simulink model "tg9"  (R2022a)
settings: Solver=ode15s  StartTime=0.0  StopTime=10  MaxStep=0.01  RelTol=1e-3
InitFcn:
  | mecha_param2
  | control_param0
values from neighbouring files (symbols this model uses):
  b0 = 0    [sim_IMMC.m]
  b1 = 1    [sim_IMMC.m]
  back0 = 0    [sim_IMMC.m]
  back1 = 0    [sim_IMMC.m]
  boff = 0    [sim_IMMC.m]
  bon = 0    [sim_IMMC.m]
  c = 0.05    [mecha_param2.m]
  c_jointstop = 0.3 / (pi/180)    (= 17.1887338539)    [mecha_param2.m]
  calctalus = sqrt((L_foot - (DJ1x_foot))^2 + (H_foot-r_cs)^2)    [mecha_param2.m]
  calctoes = sqrt((H_foot-r_cs)^2 + (DJ1x_foot)^2)    [mecha_param2.m]
  corrD = 0.001    [control_param0.m]
  DG_HAT = 0.35    [mecha_param2.m]
  DG_thigh = 0.28    [mecha_param2.m]
  DJ1x_foot = 0.16-r_cs    (= 0.135)    [mecha_param2.m]
  eref = 0.04    [mecha_param2.m]
  FmaxBFSH = 350    [mecha_param2.m]
  FmaxGAS = 1500    [mecha_param2.m]
  FmaxGLU = 1500    [mecha_param2.m]
  FmaxHAM = 3000    [mecha_param2.m]
  FmaxHFL = 2000    [mecha_param2.m]
  FmaxRF = 1200    [mecha_param2.m]
  FmaxSOL = 4000    [mecha_param2.m]
  FmaxTA = 800    [mecha_param2.m]
  FmaxVAS = 6000    [mecha_param2.m]
  g = 9.81    [mecha_param2.m]
  g0 = 0    [sim_IMMC.m]
  g1 = 0    [sim_IMMC.m]
  H_foot = 0.08    [mecha_param2.m]
  In_HAT = 3    [mecha_param2.m]
  In_shank = 0.05    [mecha_param2.m]
  In_thigh = 0.15    [mecha_param2.m]
  K = 5    [mecha_param2.m]
  knee_thigh = [0 0 -(L_thigh/2)]    [mecha_param2.m]
  Kpress = m_HAT * g / DeltaThRef    (= 104967)    [mecha_param2.m]
  L_foot = 0.2    [mecha_param2.m]
  L_HAT = 0.8    [mecha_param2.m]
  L_shank = 0.46    [mecha_param2.m]
  L_thigh = 0.46    [mecha_param2.m]
  LoHAM = table2array(mt('LoHAM', 1))    [control_param0.m]
  LoHFL = table2array(mt('LoHFL', 1))    [control_param0.m]
  longD = longD - corrD    (= 0.019)    [control_param0.m]
  loptBFSH = 0.12    [mecha_param2.m]
  loptGAS = 0.05    [mecha_param2.m]
  loptGLU = 0.11    [mecha_param2.m]
  loptHAM = 0.10    (= 0.1)    [mecha_param2.m]
  loptHFL = 0.11    [mecha_param2.m]
  loptRF = 0.08    [mecha_param2.m]
  loptSOL = 0.04    [mecha_param2.m]
  loptTA = 0.06    [mecha_param2.m]
  loptVAS = 0.08    [mecha_param2.m]
  LoTA = table2array(mt('LoTA', 1))    [control_param0.m]
  lslackBFSH = 0.10    (= 0.1)    [mecha_param2.m]
  lslackGAS = 0.40    (= 0.4)    [mecha_param2.m]
  lslackGLU = 0.13    [mecha_param2.m]
  lslackHAM = 0.31    [mecha_param2.m]
  lslackHFL = 0.10    (= 0.1)    [mecha_param2.m]
  lslackRF = 0.35    [mecha_param2.m]
  lslackSOL = 0.26    [mecha_param2.m]
  lslackTA = 0.24    [mecha_param2.m]
  lslackVAS = 0.23    [mecha_param2.m]
  m_HAT = 53.5    [mecha_param2.m]
  m_shank = 3.5    [mecha_param2.m]
  m_thigh = 8.5    [mecha_param2.m]
  midD = midD - corrD    (= 0.009)    [control_param0.m]
  N = 1.5    [mecha_param2.m]
  nonoff = 0    [control_param0.m]
  phi_a_low = (70) * (pi / 180)    (= 1.2217304764)    [mecha_param2.m]
  phi_a_up = (130) * (pi / 180)    (= 2.26892802759)    [mecha_param2.m]
  phi_dl = 180    [mecha_param2.m]
  phi_h = 230 * (pi / 180)    (= 4.01425727959)    [mecha_param2.m]
  phi_k = 175 * (pi / 180)    (= 3.05432619099)    [mecha_param2.m]
  phictoes = asind((DJ1y_foot-r_cs)/calctoes)    [mecha_param2.m]
  phimaxGASa = 100*pi/180    (= 1.74532925199)    [mecha_param2.m]
  phimaxGASk = 140*pi/180    (= 2.44346095279)    [mecha_param2.m]
  phimaxRFk = 165*pi/180    (= 2.87979326579)    [mecha_param2.m]
  phimaxSOL = 100*pi/180    (= 1.74532925199)    [mecha_param2.m]
  phimaxTA = 80*pi/180    (= 1.3962634016)    [mecha_param2.m]
  phimaxVAS = 165*pi/180    (= 2.87979326579)    [mecha_param2.m]
  phirefBFSH = 160*pi/180    (= 2.79252680319)    [mecha_param2.m]
  phirefGASa = 80*pi/180    (= 1.3962634016)    [mecha_param2.m]
  phirefGASk = 165*pi/180    (= 2.87979326579)    [mecha_param2.m]
  phirefGLU = 120*pi/180    (= 2.09439510239)    [mecha_param2.m]
  phirefHAMh = 150*pi/180    (= 2.61799387799)    [mecha_param2.m]
  phirefHAMk = 180*pi/180    (= 3.14159265359)    [mecha_param2.m]
  phirefHFL = 160*pi/180    (= 2.79252680319)    [mecha_param2.m]
  phirefRFh = 170*pi/180    (= 2.96705972839)    [mecha_param2.m]
  phirefRFk = 125*pi/180    (= 2.18166156499)    [mecha_param2.m]
  phirefSOL = 90*pi/180    (= 1.57079632679)    [mecha_param2.m]
  phirefTA = 110*pi/180    (= 1.91986217719)    [mecha_param2.m]
  phirefVAS = 120*pi/180    (= 2.09439510239)    [mecha_param2.m]
  phiScaleGASa = acos(rGASamin/rGASamax)/(phiminGASa-phimaxGASa)    [mecha_param2.m]
  phiScaleGASk = acos(rGASkmin/rGASkmax)/(phiminGASk-phimaxGASk)    [mecha_param2.m]
  phiScaleRFk = acos(rRFkmin/rRFkmax)/(phiminRFk-phimaxRFk)    [mecha_param2.m]
  phiScaleSOL = acos(rSOLmin/rSOLmax)/(phiminSOL-phimaxSOL)    [mecha_param2.m]
  phiScaleTA = acos(rTAmin/rTAmax)/(phiminTA-phimaxTA)    [mecha_param2.m]
  phiScaleVAS = acos(rVASmin/rVASmax)/(phiminVAS-phimaxVAS)    [mecha_param2.m]
  r1 = 0    [sim_IMMC.m]
  r_cs = 0.025    [mecha_param2.m]
  rBFSH = 0.04    [mecha_param2.m]
  rGASamax = 0.06    [mecha_param2.m]
  rGASkmax = 0.05    [mecha_param2.m]
  rGLU = 0.08    [mecha_param2.m]
  rHAMh = 0.08    [mecha_param2.m]
  rHAMk = 0.05    [mecha_param2.m]
  rHFL = 0.08    [mecha_param2.m]
  rhoBFSH = 0.7    [mecha_param2.m]
  rhoGASa = 0.7    [mecha_param2.m]
  rhoGASk = 0.7    [mecha_param2.m]
  rhoGLU = 0.5    [mecha_param2.m]
  rhoHAMh = 0.5    [mecha_param2.m]
  rhoHAMk = 0.5    [mecha_param2.m]
  rhoHFL = 0.5    [mecha_param2.m]
  rhoRFh = 0.3    [mecha_param2.m]
  rhoRFk = 0.5    [mecha_param2.m]
  rhoSOL = 0.5    [mecha_param2.m]
  rhoTA = 0.7    [mecha_param2.m]
  rhoVAS = 0.6    [mecha_param2.m]
  rRFh = 0.08    [mecha_param2.m]
  rRFkmax = 0.06    [mecha_param2.m]
  rSOLmax = 0.06    [mecha_param2.m]
  ... (+25 more)
undefined symbols (not defined in the file or in its folder): beta11, beta12, beta13, beta14, beta15, beta16, beta21, beta22, beta23, beta24, beta25, beta26, beta31, beta32, beta33, beta34, beta35, beta36, beta41, beta42, beta43, beta44, beta45, beta46, beta51, beta52, beta53, beta54, beta55, beta56, betab1, betab2, betab3, betab4, betab5, betab6, betap11, betap12, betap13, betap14, betap15, betap16, betap21, betap22, betap23, betap24, betap25, betap26, betap31, betap32, betap33, betap34, betap35, betap36, betap41, betap42, betap43, betap44, betap45, betap46 ... (+102)
libraries: sm_lib x89, simulink x72, nesl_utility x58, simulink_extras x18
(part 3 of 12)

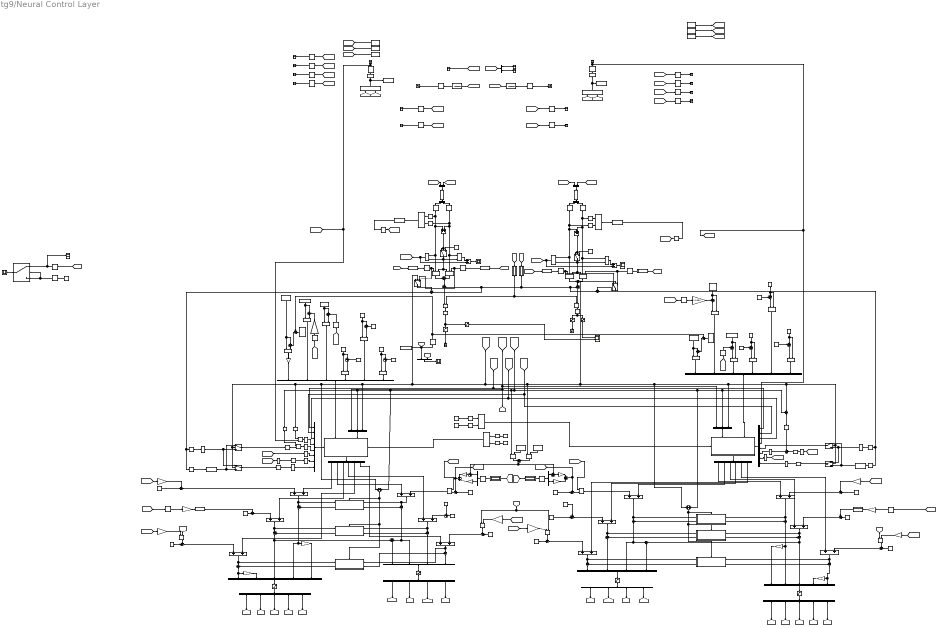
== system tg9/Neural Control Layer ==
  note: Reference left muscles length
  note: NEURAL CONTROL LAYER
  note: Reference right muscles length
  note: Stance phase left force/length inputs
  note: Stance phase right force/length inputs
  AHipExt : Constant  Value=0
  AHipExt1 : Constant  Value=0
  AHipFlexL{,1..4} (5 alike) : Constant  Value=0
  AHipFlexR : Constant  Value=0
  AankleExt : Constant  Value=0
  AankleExt1 : Constant  Value=0
  AankleFlexL : Constant  Value=0
  Add1 : Sum  Inputs=+-
  Add10 : Sum
  Add3 : Sum  Inputs=+-
  Add8 : Sum
  AkneeExt : Constant  Value=0
  AkneeExt1 : Constant  Value=0
  AkneeFlexL : Constant  Value=0
  AkneeFlexL1 : Constant  Value=0
  AkneeFlexR : Constant  Value=0
  AkneeFlexR1 : Constant  Value=0
  AnkleFlexR : Constant  Value=0
  Body Pitch Velocity Sense delay : TransportDelay  DelayTime=shortD  BufferSize=2048
  Body Pitch Velocity Sense delay1 : TransportDelay  DelayTime=shortD  BufferSize=2048
  Cast To Double{,1,3..4} (4 alike) : DataTypeConversion  OutDataTypeStr=double  SaturateOnIntegerOverflow=off  RndMeth=Floor
  Compare To Constant{2..5} (4 alike) : simulink/Logic and Bit Operations/Compare To Constant  relop=>  const=20  OutDataTypeStr=boolean  ZeroCross=off
  Constant1 : Constant  Value=LoHAM
  Constant20 : Constant  Value=LoHAM
  Constant21 : Constant  Value=LoTA
  Constant22 : Constant  Value=LoHFL
  Constant3 : Constant  Value=10
  Constant4 : Constant  Value=10
  Constant5 : Constant  Value=LoTA
  Constant6 : Constant  Value=LoHFL
  Data Type Conversion{,1..13} (14 alike) : DataTypeConversion  OutDataTypeStr=double  SaturateOnIntegerOverflow=off  RndMeth=Floor
  Demux{,3,9..11} (5 alike) : Demux  Outputs=2
  Demux23 : Demux  Outputs=6
  Demux4 : Demux  Outputs=5
  Demux5 : Demux
  Demux6 : Demux  Outputs=6
  Demux7 : Demux  Outputs=5
  Demux8 : Demux
  Divide : Product  Inputs=**/
  Divide1 : Product  Inputs=/**
  Divide{2..5,10..14,19,21,24} (12 alike) : Product  Inputs=*/
  Divide{15..17,25} (4 alike) : Product  Inputs=**
  Divide{8..9,18,20,22..23} (6 alike) : Product  Inputs=/*
  Divide6 : Product  Inputs=**/
  Divide7 : Product  Inputs=/**
  F-S{1..6,11} (7 alike) : Constant  Value=0  OutDataTypeStr=Inherit: Inherit via back propagation
  Gain : Gain
  Gain3 : Gain  Gain=modham
  Gain4 : Gain  Gain=modgas
  Gain5 : Gain  Gain=1/1350
  Gain61 : Gain  Gain=modham
  Gain62 : Gain  Gain=modgas
  Gain9 : Gain  Gain=1/1350
  Hip joint sense delay : TransportDelay  DelayTime=shortD  BufferSize=2048
  Hip joint sense delay1 : TransportDelay  DelayTime=shortD  BufferSize=2048
  Hit Crossing{,1..5,7..8} (8 alike) : HitCross  HitCrossingOffset=0.5  HitCrossingDirection=rising  ZeroCross=off
  IMsLeft : Subsystem
      settings: PortSchema="{\"entries\":[{\"content\":{\"sides\":[{\"content\":{\"connectorIds\":[\"In1\"]},\"type\":\"ConnectorPlacement.EquallySpacedRectSide\",\"uuid\":\"2c5d9d99-aee6-47ec-aaeb-adda6ea14088\"},{\"content\":{\"connectorIds\":[\"In4\"],\"side\":\"RIGHT\"},\"type\":\"ConnectorPlacement.EquallySpacedRectSide\",\"uuid\":\"43d4876d-2238-4aaf-9da2-83035815f60d\"},{\"content\":{\"connectorIds\":[\"In2\",\"In3\"],\"side\":\"TOP\"},\"type\":\"ConnectorPlacement.EquallySpacedRectSide\",\"uuid\":\"a1006f79-6931-4ab8-841c-7153832dea90\"},{\"content\":{\"connectorIds\":[\"Out1\"],\"side\":\"BOTTOM\"},\"type\":\"ConnectorPlacement.EquallySpacedRectSide\",\"uuid\":\"458ab36f-15e6-408a-9bf0-13c7ce18e979\"}]},\"type\":\"ConnectorPlacement.EquallySpacedConnector\",\"uuid\":\"44ba4de4-75d8-42cf-8d5d-6a448bd4d886\"}],\"packageUris\":[\"http://schema.mathworks.com/mf0/Connector/R2020b\"],\"version\":\"1.0\"}"
  IMsRight : Subsystem
      settings: PortSchema="{\"entries\":[{\"content\":{\"sides\":[{\"content\":{\"connectorIds\":[\"In1\"]},\"type\":\"ConnectorPlacement.EquallySpacedRectSide\",\"uuid\":\"2c5d9d99-aee6-47ec-aaeb-adda6ea14088\"},{\"content\":{\"connectorIds\":[\"In4\"],\"side\":\"RIGHT\"},\"type\":\"ConnectorPlacement.EquallySpacedRectSide\",\"uuid\":\"43d4876d-2238-4aaf-9da2-83035815f60d\"},{\"content\":{\"connectorIds\":[\"In2\",\"In3\"],\"side\":\"TOP\"},\"type\":\"ConnectorPlacement.EquallySpacedRectSide\",\"uuid\":\"a1006f79-6931-4ab8-841c-7153832dea90\"},{\"content\":{\"connectorIds\":[\"Out1\"],\"side\":\"BOTTOM\"},\"type\":\"ConnectorPlacement.EquallySpacedRectSide\",\"uuid\":\"458ab36f-15e6-408a-9bf0-13c7ce18e979\"}]},\"type\":\"ConnectorPlacement.EquallySpacedConnector\",\"uuid\":\"44ba4de4-75d8-42cf-8d5d-6a448bd4d886\"}],\"packageUris\":[\"http://schema.mathworks.com/mf0/Connector/R2020b\"],\"version\":\"1.0\"}"
  IsPositive{,1..5} (6 alike) : simulink/Logic and Bit Operations/Compare To Zero  relop=>  OutDataTypeStr=boolean  ZeroCross=off
  IsPositive6 : simulink/Logic and Bit Operations/Compare To Zero  relop=<  OutDataTypeStr=boolean  ZeroCross=off
  IsPositive7 : simulink/Logic and Bit Operations/Compare To Zero  relop=<  OutDataTypeStr=boolean  ZeroCross=off
  KAnkleExt : Gain  Gain=KAnkleExt
  KAnkleExt1 : Gain  Gain=KAnkleExt
  KAnkleFlex : Gain  Gain=KAnkleFlex
  KAnkleFlex1 : Gain  Gain=KAnkleFlex
  KHipExt : Gain  Gain=KHipExt
  KHipExt1 : Gain  Gain=KHipExt
  KKneeExt : Gain  Gain=KKneeExt
  KKneeExt1 : Gain  Gain=KKneeExt
  Kq : Gain  Gain=Kq
  Kq1 : Gain  Gain=Kq
  Kw : Gain  Gain=Kw
  Kw1 : Gain  Gain=Kw
  L GAS golgi delay : TransportDelay  DelayTime=longD  BufferSize=2048
  L GLU golgi delay : TransportDelay  DelayTime=shortD  BufferSize=2048
  L HAM golgi delay : TransportDelay  DelayTime=shortD  BufferSize=2048
  L HAM spindle delay : TransportDelay  DelayTime=shortD  BufferSize=2048
  "L HFL spindle delay " : TransportDelay  DelayTime=shortD  BufferSize=2048
  L SOL golgi delay : TransportDelay  DelayTime=longD  BufferSize=2048
  L SOL golgi delay1 : TransportDelay  DelayTime=shortD  BufferSize=2048
  L Skin Load Sensor delay : TransportDelay  DelayTime=midD  BufferSize=2048
  L Skin Load Sensor delay{1..8} (8 alike) : TransportDelay  DelayTime=longD  BufferSize=2048
  L TA spindle delay : TransportDelay  DelayTime=longD  BufferSize=2048
  L Thigh Sensor delay : TransportDelay  DelayTime=shortD  BufferSize=2048
  L Thigh Sensor delay1 : TransportDelay  DelayTime=shortD  BufferSize=2048
  L VAS golgi delay : TransportDelay  DelayTime=midD  BufferSize=2048
  Left Stance : Logic  Operator=OR  AllPortsSameDT=off
  Logical Operator : Logic  Operator=NOT  AllPortsSameDT=off  OutDataTypeStr=boolean
  Logical Operator{1..3,5..7} (6 alike) : Logic  Operator=OR  AllPortsSameDT=off  OutDataTypeStr=boolean
  Logical Operator4 : Logic  Operator=NOT  AllPortsSameDT=off  OutDataTypeStr=boolean
  Mux : Mux  Inputs=2
  Mux1 : Mux  Inputs=5
  Mux10 : Mux  Inputs=2
  Mux11 : Mux  Inputs=3
  Mux12 : Mux  Inputs=3
  Mux14 : Mux  Inputs=6
  Mux15 : Mux  Inputs=8
  Mux4 : Mux
  Mux5 : Mux  Inputs=8
  Mux6 : Mux  Inputs=6
  Mux7 : Mux  Inputs=5
  Mux8 : Mux
  Mux9 : Mux  Inputs=2
  Product{,1..3} (4 alike) : Product
  R GAS golgi delay : TransportDelay  DelayTime=longD  BufferSize=2048
  R GLU golgi delay : TransportDelay  DelayTime=shortD  BufferSize=2048
  R HAM golgi delay : TransportDelay  DelayTime=shortD  BufferSize=2048
  R HAM spindle delay : TransportDelay  DelayTime=shortD  BufferSize=2048
  R HFL spindle delay : TransportDelay  DelayTime=shortD  BufferSize=2048
  R SOL golgi delay : TransportDelay  DelayTime=longD  BufferSize=2048
  R Skin Load Sensor delay : TransportDelay  DelayTime=midD  BufferSize=2048
  R TA spindle delay : TransportDelay  DelayTime=longD  BufferSize=2048
  R VAS golgi delay : TransportDelay  DelayTime=midD  BufferSize=2048
  Right Stance : Logic  Operator=OR  AllPortsSameDT=off
  Saturation : Saturate  UpperLimit=0  LowerLimit=-inf  ZeroCross=off
  Saturation1 : Saturate  UpperLimit=inf  LowerLimit=0  ZeroCross=off
  Saturation{2..5} (4 alike) : Saturate  UpperLimit=1  LowerLimit=0.01  ZeroCross=off
  Saturation6 : Saturate  UpperLimit=0  LowerLimit=-inf  ZeroCross=off
  Saturation7 : Saturate  UpperLimit=inf  LowerLimit=0  ZeroCross=off
  Scope : Scope
  Scope1 : Scope
  Scope5 : Scope
  Subsystem1 : Subsystem
      settings: PortSchema="{\"entries\":[{\"content\":{\"sides\":[{\"content\":{\"connectorIds\":[\"In1\",\"Out2\"]},\"type\":\"ConnectorPlacement.EquallySpacedRectSide\",\"uuid\":\"6fc3d8a1-10cd-49a3-bec6-ab71dc5c57d9\"},{\"content\":{\"connectorIds\":[\"In3\",\"Out1\"],\"side\":\"RIGHT\"},\"type\":\"ConnectorPlacement.EquallySpacedRectSide\",\"uuid\":\"bd27b384-a872-48d3-89d5-92190537daea\"},{\"content\":{\"connectorIds\":[\"In2\"],\"side\":\"TOP\"},\"type\":\"ConnectorPlacement.EquallySpacedRectSide\",\"uuid\":\"3f5f6709-2670-4a61-8889-7ddb002f3d5b\"}]},\"type\":\"ConnectorPlacement.EquallySpacedConnector\",\"uuid\":\"7b4a72ad-30b2-4cc1-b684-e51201412c74\"}],\"packageUris\":[\"http://schema.mathworks.com/mf0/Connector/R2020b\"],\"version\":\"1.0\"}"
  Subsystem2 : Subsystem
      settings: PortSchema="{\"entries\":[{\"content\":{\"sides\":[{\"content\":{\"connectorIds\":[\"In1\",\"Out2\"]},\"type\":\"ConnectorPlacement.EquallySpacedRectSide\",\"uuid\":\"6fc3d8a1-10cd-49a3-bec6-ab71dc5c57d9\"},{\"content\":{\"connectorIds\":[\"In3\",\"Out1\"],\"side\":\"RIGHT\"},\"type\":\"ConnectorPlacement.EquallySpacedRectSide\",\"uuid\":\"bd27b384-a872-48d3-89d5-92190537daea\"},{\"content\":{\"connectorIds\":[\"In2\"],\"side\":\"TOP\"},\"type\":\"ConnectorPlacement.EquallySpacedRectSide\",\"uuid\":\"3f5f6709-2670-4a61-8889-7ddb002f3d5b\"}]},\"type\":\"ConnectorPlacement.EquallySpacedConnector\",\"uuid\":\"7b4a72ad-30b2-4cc1-b684-e51201412c74\"}],\"packageUris\":[\"http://schema.mathworks.com/mf0/Connector/R2020b\"],\"version\":\"1.0\"}"
  Subsystem3 : Subsystem
      settings: PortSchema="{\"entries\":[{\"content\":{\"sides\":[{\"content\":{\"connectorIds\":[\"In1\",\"Out2\"]},\"type\":\"ConnectorPlacement.EquallySpacedRectSide\",\"uuid\":\"6fc3d8a1-10cd-49a3-bec6-ab71dc5c57d9\"},{\"content\":{\"connectorIds\":[\"In3\",\"Out1\"],\"side\":\"RIGHT\"},\"type\":\"ConnectorPlacement.EquallySpacedRectSide\",\"uuid\":\"bd27b384-a872-48d3-89d5-92190537daea\"},{\"content\":{\"connectorIds\":[\"In2\"],\"side\":\"TOP\"},\"type\":\"ConnectorPlacement.EquallySpacedRectSide\",\"uuid\":\"3f5f6709-2670-4a61-8889-7ddb002f3d5b\"}]},\"type\":\"ConnectorPlacement.EquallySpacedConnector\",\"uuid\":\"7b4a72ad-30b2-4cc1-b684-e51201412c74\"}],\"packageUris\":[\"http://schema.mathworks.com/mf0/Connector/R2020b\"],\"version\":\"1.0\"}"
  Subsystem4 : Subsystem
      settings: PortSchema="{\"entries\":[{\"content\":{\"sides\":[{\"content\":{\"connectorIds\":[\"In1\",\"Out2\"]},\"type\":\"ConnectorPlacement.EquallySpacedRectSide\",\"uuid\":\"6fc3d8a1-10cd-49a3-bec6-ab71dc5c57d9\"},{\"content\":{\"connectorIds\":[\"In3\",\"Out1\"],\"side\":\"RIGHT\"},\"type\":\"ConnectorPlacement.EquallySpacedRectSide\",\"uuid\":\"bd27b384-a872-48d3-89d5-92190537daea\"},{\"content\":{\"connectorIds\":[\"In2\"],\"side\":\"TOP\"},\"type\":\"ConnectorPlacement.EquallySpacedRectSide\",\"uuid\":\"3f5f6709-2670-4a61-8889-7ddb002f3d5b\"}]},\"type\":\"ConnectorPlacement.EquallySpacedConnector\",\"uuid\":\"7b4a72ad-30b2-4cc1-b684-e51201412c74\"}],\"packageUris\":[\"http://schema.mathworks.com/mf0/Connector/R2020b\"],\"version\":\"1.0\"}"
  Subsystem5 : Subsystem
      settings: PortSchema="{\"entries\":[{\"content\":{\"sides\":[{\"content\":{\"connectorIds\":[\"In1\",\"Out2\"]},\"type\":\"ConnectorPlacement.EquallySpacedRectSide\",\"uuid\":\"6fc3d8a1-10cd-49a3-bec6-ab71dc5c57d9\"},{\"content\":{\"connectorIds\":[\"In3\",\"Out1\"],\"side\":\"RIGHT\"},\"type\":\"ConnectorPlacement.EquallySpacedRectSide\",\"uuid\":\"bd27b384-a872-48d3-89d5-92190537daea\"},{\"content\":{\"connectorIds\":[\"In2\"],\"side\":\"TOP\"},\"type\":\"ConnectorPlacement.EquallySpacedRectSide\",\"uuid\":\"3f5f6709-2670-4a61-8889-7ddb002f3d5b\"}]},\"type\":\"ConnectorPlacement.EquallySpacedConnector\",\"uuid\":\"7b4a72ad-30b2-4cc1-b684-e51201412c74\"}],\"packageUris\":[\"http://schema.mathworks.com/mf0/Connector/R2020b\"],\"version\":\"1.0\"}"
  Subsystem6 : Subsystem
      settings: PortSchema="{\"entries\":[{\"content\":{\"sides\":[{\"content\":{\"connectorIds\":[\"In1\",\"Out2\"]},\"type\":\"ConnectorPlacement.EquallySpacedRectSide\",\"uuid\":\"6fc3d8a1-10cd-49a3-bec6-ab71dc5c57d9\"},{\"content\":{\"connectorIds\":[\"In3\",\"Out1\"],\"side\":\"RIGHT\"},\"type\":\"ConnectorPlacement.EquallySpacedRectSide\",\"uuid\":\"bd27b384-a872-48d3-89d5-92190537daea\"},{\"content\":{\"connectorIds\":[\"In2\"],\"side\":\"TOP\"},\"type\":\"ConnectorPlacement.EquallySpacedRectSide\",\"uuid\":\"3f5f6709-2670-4a61-8889-7ddb002f3d5b\"}]},\"type\":\"ConnectorPlacement.EquallySpacedConnector\",\"uuid\":\"7b4a72ad-30b2-4cc1-b684-e51201412c74\"}],\"packageUris\":[\"http://schema.mathworks.com/mf0/Connector/R2020b\"],\"version\":\"1.0\"}"
  Sum{,7,18..19,22..23,25,30} (8 alike) : Sum  Inputs=+|+
  Sum{10..11,38..39,42,49..50} (7 alike) : Sum  Inputs=|++
  Sum{5..6,9,12..13,20,24,26..27,31..35,40..41,51..57} (23 alike) : Sum  Inputs=++|
  Sum{3,8,14,16,28,36,48} (7 alike) : Sum  Inputs=|+-
  Sum{4,15,17,21,29,37,44,46..47} (9 alike) : Sum  Inputs=-+|
  Sum43 : Sum  Inputs=+|||+
  Switch : Switch  Criteria=u2 > Threshold  ZeroCross=off  SaturateOnIntegerOverflow=off  InputSameDT=off
  Switch1 : Switch  Criteria=u2 > Threshold  Threshold=10  ZeroCross=off  SaturateOnIntegerOverflow=off  InputSameDT=off
  Switch2 : Switch  Criteria=u2 > Threshold  Threshold=10  ZeroCross=off  SaturateOnIntegerOverflow=off  InputSameDT=off
  Switch{3..8} (6 alike) : Switch  Criteria=u2 ~= 0  ZeroCross=off  SaturateOnIntegerOverflow=off  InputSameDT=off
  Terminator{1..2,4..5,7..8,10,12..13,15,17,19..28} (21 alike) : Terminator
  To Workspace1 : ToWorkspace  VariableName=Rcontact  SampleTime=-1
  To Workspace7 : ToWorkspace  VariableName=theta  SampleTime=-1
  To Workspace85 : ToWorkspace  VariableName=Lcontact  SampleTime=-1
  Transfer Fcn : TransferFcn  Denominator=[0.02 1]
  Transfer Fcn1 : TransferFcn  Denominator=[0.02 1]
  Trigonometric Function : Trigonometry  Operator=atan
  Trigonometric Function1 : Trigonometry  Operator=atan
  knee pain delay : TransportDelay  DelayTime=midD  BufferSize=2048
  knee pain delay R : TransportDelay  DelayTime=midD  BufferSize=2048
  lambda-null3L : Constant  Value=15  OutDataTypeStr=Inherit: Inherit via back propagation
  lambda-null3R : Constant  Value=15  OutDataTypeStr=Inherit: Inherit via back propagation
  lambda-null4L : Constant  Value=0.75  OutDataTypeStr=Inherit: Inherit via back propagation
  lambda-null4R : Constant  Value=0.75  OutDataTypeStr=Inherit: Inherit via back propagation
  lambda-null5L : Constant  Value=15  OutDataTypeStr=Inherit: Inherit via back propagation
  lambda-null5R : Constant  Value=15  OutDataTypeStr=Inherit: Inherit via back propagation
  lambda-s1L : Constant  Value=lambda_s1  OutDataTypeStr=Inherit: Inherit via back propagation
  lambda-s1R : Constant  Value=lambda_s1  OutDataTypeStr=Inherit: Inherit via back propagation
  lambda-s2L : Constant  Value=lambda_s2  OutDataTypeStr=Inherit: Inherit via back propagation
  lambda-s2R : Constant  Value=lambda_s2  OutDataTypeStr=Inherit: Inherit via back propagation
  lambdaxL : Constant  Value=lambdax
  lambdaxR : Constant  Value=lambdax
  lean_ref : Constant  Value=lean_ref
  lenf_ref : Constant  Value=lean_ref
  motorpoolL{1..6} (6 alike) : Sum
  motorpoolR{1..6} (6 alike) : Sum
  noisy : Subsystem
  noisy1 : Subsystem
  noisy10 : Subsystem
  noisy11 : Subsystem
  noisy2 : Subsystem
  noisy3 : Subsystem
  noisy4 : Subsystem
  noisy5 : Subsystem
  noisy6 : Subsystem
  noisy7 : Subsystem
  noisy8 : Subsystem
  noisy9 : Subsystem
  thetabo : Constant  Value=lean_ref_back
  thetao : Constant  Value=lean_ref
  xForce : Scope
  xForce1 : Scope
  xForce2 : Scope  NumInputPorts=2
  tag scope: LBFSHstim=global, LGASstim=global, LGLUstim=global, LHAMstim=global, LHFLstim=global, LRFstim=global, LSOLstim=global, LTAstim=global, LVASstim=global, LyHAM=global, LyHFL=global, LyTA=global, RBFSHstim=global, RGASstim=global, RGLUstim=global, RHAMstim=global, RHFLstim=global, RRFstim=global, RSOLstim=global, RTAstim=global, RVASstim=global, RyHAM=global, RyHFL=global, RyTA=global
  wires:
  [LGASgolgi] -> L GAS golgi delay/1
  Constant1/1 -> [LyHAM]
  Constant5/1 -> [LyTA]
  Constant6/1 -> [LyHFL]
  Constant22/1 -> [RyHFL]
  Constant21/1 -> [RyTA]
  [LTAspindle] -> L TA spindle delay/1
  Constant20/1 -> [RyHAM]
  [LVASgolgi] -> L VAS golgi delay/1
  [Ldx] -> Transfer Fcn/1
  [LHFLspindle] -> "L HFL spindle delay "/1
  [LHAMspindle] -> L HAM spindle delay/1
  [LHAMgolgi] -> L HAM golgi delay/1
  [LGLUgolgi] -> L GLU golgi delay/1
  [LballContact] -> Left Stance/1
  [LheelContact] -> Left Stance/2
  Data Type Conversion/1 -> L Skin Load Sensor delay/1
  Left Stance/1 -> To Workspace85/1, Data Type Conversion/1
  [RballContact] -> Right Stance/1
  [RheelContact] -> Right Stance/2
  Data Type Conversion1/1 -> R Skin Load Sensor delay/1
  Right Stance/1 -> To Workspace1/1, Data Type Conversion1/1
  [Rdx] -> Transfer Fcn1/1
  Transfer Fcn/1 -> L Thigh Sensor delay/1
  Transfer Fcn1/1 -> L Thigh Sensor delay1/1
  L Thigh Sensor delay1/1 -> Terminator4/1
  [LKneeState] -> Terminator5/1
  L Thigh Sensor delay/1 -> Terminator8/1
  [RVASgolgi] -> R VAS golgi delay/1
  [RGASgolgi] -> R GAS golgi delay/1
  [RTAspindle] -> R TA spindle delay/1
  [RKneeState] -> Demux3/1
  [RHFLspindle] -> R HFL spindle delay/1
  [RHAMspindle] -> R HAM spindle delay/1
  [RHAMgolgi] -> R HAM golgi delay/1
  [RGLUgolgi] -> R GLU golgi delay/1
  L VAS golgi delay/1 -> Gain5/1
  L GAS golgi delay/1 -> Terminator10/1
  L TA spindle delay/1 -> Terminator12/1
  R VAS golgi delay/1 -> Gain9/1
  R GAS golgi delay/1 -> Terminator15/1
  R TA spindle delay/1 -> Terminator17/1
  R HFL spindle delay/1 -> Terminator19/1
  R HAM spindle delay/1 -> Terminator20/1
  R HAM golgi delay/1 -> Terminator21/1
  R GLU golgi delay/1 -> Terminator22/1
  "L HFL spindle delay "/1 -> Terminator23/1
  L HAM spindle delay/1 -> Terminator24/1
  L HAM golgi delay/1 -> Terminator25/1
  L GLU golgi delay/1 -> Terminator26/1
  [ankleL_control] -> KAnkleFlex/1
  Subsystem2/1(Out1) -> Sum17/1
  motorpoolL5/1 -> Subsystem2/1(In1), Sum16/1
  Subsystem2/2(Out2) -> Sum16/2
  motorpoolL2/1 -> Subsystem3/3(In2), Sum15/2
  Sum6/1 -> motorpoolL5/1
  motorpoolL6/1 -> Subsystem2/3(In2), Sum17/2
  Sum11/1 -> Divide12/2
  Sum7/1 -> [ExtHipLControl], Sum20/1
  [ExtHipLControl] -> KHipExt/1
  Subsystem3/2(Out2) -> Sum14/2
  Sum10/1 -> Divide10/2
  Subsystem3/1(Out1) -> Sum15/1
  motorpoolL1/1 -> Subsystem3/1(In1), Sum14/1
  Divide12/1 -> Mux6/4
  Add10/1 -> Switch1/1, Switch1/2
  lambda-null3R/1 -> Divide12/1, Sum11/1
  lambda-s2L/1 -> Sum10/1, Divide10/1
  Sum36/1 -> Sum18/1, Mux7/3
  Mux7/1 -> Saturation2/1
  Saturation2/1 -> Demux7/1
  Demux7/4 -> [LGLUstim]
  Saturation3/1 -> Demux8/1
  Mux8/1 -> Saturation3/1
  Sum17/1 -> Mux8/4
  Demux8/2 -> [LHFLstim]
  [dy] -> Body Pitch Velocity Sense delay1/1
  Body Pitch Velocity Sense delay/1 -> Switch/3, Switch/2
  Body Pitch Velocity Sense delay1/1 -> Scope5/1, Switch/1
  Switch/1 -> Scope1/1
  noisy2/1(Out1) -> L Skin Load Sensor delay4/1
  noisy1/1(Out1) -> L Skin Load Sensor delay3/1
  Divide/1 -> Sum/1
  Divide1/1 -> Sum/2
  L Skin Load Sensor delay1/1 -> Compare To Constant2/1, Divide/2, Divide3/1, Add10/1
  L Skin Load Sensor delay2/1 -> Compare To Constant3/1, Divide1/2, Divide4/1, Add10/2
  L Skin Load Sensor delay3/1 -> Divide1/3, Switch7/3
  L Skin Load Sensor delay4/1 -> Switch7/1, Divide/1
  Sum3/1 -> Divide2/1
  Trigonometric Function/1 -> Saturation/1, Saturation1/1
  [FRheel] -> Mux9/2
  [FRball] -> Mux9/1
  Constant3/1 -> Switch1/3
  Sum/1 -> Sum3/1
  Switch1/1 -> Divide/3, Divide1/1, Divide4/2, Divide3/2
  Divide10/1 -> Mux6/3
  Demux7/1 -> [LSOLstim]
  Demux7/3 -> [LVASstim]
  AankleExt/1 -> Sum6/2
  [ankleL_control] -> KAnkleExt/1
  Divide3/1 -> [ankleL_control], Add1/2
  Divide4/1 -> Add1/1
  Add1/1 -> xForce/1
  Demux/2 -> Kw/1
  Kw/1 -> Sum7/2
  Hip joint sense delay/1 -> Demux/1
  Kq/1 -> Sum7/1
  Compare To Constant2/1 -> Logical Operator1/1
  Compare To Constant3/1 -> Logical Operator1/2
  Logical Operator1/1 -> Cast To Double/1
  Sum37/1 -> Mux8/3
  Demux8/3 -> [LBFSHstim]
  Sum14/1 -> Mux7/4, Gain3/1
  Demux7/2 -> [LGASstim]
  Demux7/5 -> [LHAMstim]
  AHipExt/1 -> Sum12/2
  KHipExt/1 -> Sum12/1
  AankleFlexL/1 -> Sum13/2
  AHipFlexL/1 -> Sum20/2
  Divide15/1 -> motorpoolL2/2
  Demux4/5 -> [RSOLstim]
  Demux4/2 -> [RGLUstim]
  Sum4/1 -> Mux1/2, Gain61/1
  Demux5/2 -> [RBFSHstim]
  Sum48/1 -> Mux4/2
  Demux4/3 -> [RVASstim]
  Demux4/1 -> [RHAMstim]
  Demux5/3 -> [RHFLstim]
  Demux5/1 -> [RTAstim]
  Sum8/1 -> Mux4/3, Sum19/1
  Mux4/1 -> Saturation5/1
  Saturation5/1 -> Demux5/1
  Demux4/4 -> [RGASstim]
  Saturation4/1 -> Demux4/1
  Mux1/1 -> Saturation4/1
  Sum47/1 -> Mux1/3, Sum19/2
  motorpoolR1/1 -> Subsystem6/3(In2), Sum4/2
  Subsystem6/2(Out2) -> Sum8/2
  Subsystem6/1(Out1) -> Sum4/1
  motorpoolR6/1 -> Sum28/1, Subsystem5/1(In1)
  motorpoolR2/1 -> Sum8/1, Subsystem6/1(In1)
  Subsystem5/1(Out1) -> Sum21/1
  motorpoolR5/1 -> Sum21/2, Subsystem5/3(In2)
  Subsystem5/2(Out2) -> Sum28/2
  lambda-null4L/1 -> Sum27/2, Divide20/2
  Sum27/1 -> Divide20/1
  lambda-null5L/1 -> Divide18/2, Sum26/2
  F-S1/1 -> Sum26/1
  Divide18/1 -> Mux14/6
  Sum26/1 -> Divide18/1
  [x] -> noisy/1(In1)
  [xLball] -> noisy2/1(In1)
  noisy3/1(Out1) -> Hip joint sense delay/1
  Mux/1 -> noisy5/1(In1)
  noisy5/1(Out1) -> Demux9/1
  Demux9/1 -> L Skin Load Sensor delay1/1
  Demux9/2 -> L Skin Load Sensor delay2/1
  [FLball] -> Mux/1
  [FLheel] -> Mux/2
  Sum28/1 -> Mux4/1
  Demux10/2 -> L Skin Load Sensor delay6/1
  Demux10/1 -> L Skin Load Sensor delay5/1
  noisy10/1(Out1) -> Demux10/1
  Mux9/1 -> noisy10/1(In1)
  Compare To Constant5/1 -> Logical Operator3/2
  Compare To Constant4/1 -> Logical Operator3/1
  Add3/1 -> xForce1/1
  Divide14/1 -> Add3/1
  Divide13/1 -> Add3/2, [ankleR_control]
  Switch2/1 -> Divide7/1, Divide6/3, Divide14/2, Divide13/2
  Sum22/1 -> Sum29/2
  Constant4/1 -> Switch2/3
  Sum29/1 -> Divide8/2
  L Skin Load Sensor delay8/1 -> Switch8/1, Divide6/1
  L Skin Load Sensor delay7/1 -> Divide7/3, Switch8/3
  L Skin Load Sensor delay5/1 -> Add8/1, Divide6/2, Divide13/1, Compare To Constant5/1
  Divide7/1 -> Sum22/2
  Divide6/1 -> Sum22/1
  noisy8/1(Out1) -> L Skin Load Sensor delay7/1
  noisy9/1(Out1) -> L Skin Load Sensor delay8/1
  Divide2/1 -> Trigonometric Function/1
  [y] -> noisy6/1(In1)
  Divide8/1 -> Trigonometric Function1/1
  Trigonometric Function1/1 -> Saturation6/1, Saturation7/1
  Logical Operator3/1 -> Cast To Double1/1
  Cast To Double1/1 -> Logical Operator/1
  noisy7/1(Out1) -> Hip joint sense delay1/1
  Hip joint sense delay1/1 -> Demux11/1
  Kw1/1 -> Sum30/2
  Demux11/2 -> Kw1/1
  AHipFlexR/1 -> Sum31/2
  Divide16/1 -> motorpoolR2/1
  Sum44/1 -> IsPositive6/1, IsPositive/1
  AnkleFlexR/1 -> Sum32/2
  [ankleR_control] -> KAnkleFlex1/1
  KHipExt1/1 -> Sum33/1
  AankleExt1/1 -> Sum35/2
  AHipExt1/1 -> Sum33/2
  Sum33/1 -> motorpoolR1/2
  R Skin Load Sensor delay/1 -> Mux15/4, [Rhipc], Terminator27/1
  [ankleR_control] -> KAnkleExt1/1
  Sum30/1 -> [ExtHipRControl], Sum31/1
  [ExtHipRControl] -> KHipExt1/1
  [xRball] -> noisy9/1(In1)
  [xLheel] -> noisy1/1(In1)
  Sum12/1 -> motorpoolL1/1
  Sum32/1 -> motorpoolR6/1
  Sum35/1 -> motorpoolR5/2
  Saturation/1 -> Terminator7/1
  Saturation6/1 -> Terminator13/1
  Mux6/1 -> IMsLeft/2(eta)
  Mux11/1 -> IMsLeft/3(drivers)
  Mux14/1 -> IMsRight/3(eta)
  Divide5/1 -> Mux6/5
  Divide19/1 -> Mux6/6
  lambda-null4R/1 -> Sum38/1, Divide5/1
  Sum38/1 -> Divide5/2
  Sum39/1 -> Divide19/2
  F-S5/1 -> Sum39/2
  lambda-null5R/1 -> Divide19/1, Sum39/1
  Divide20/1 -> Mux14/5
  Divide22/1 -> Mux14/4
  Sum40/1 -> Divide22/1
  lambda-null3L/1 -> Divide22/2, Sum40/2
  lambda-s2R/1 -> Divide23/2, Sum41/2
  Sum41/1 -> Divide23/1
  R SOL golgi delay/1 -> Sum41/1
  Divide23/1 -> Mux14/3
  Mux5/1 -> IMsLeft/1(triggers)
  Mux15/1 -> IMsRight/4(triggers)
  Hit Crossing7/1 -> Data Type Conversion11/1
  [Rhipc] -> Data Type Conversion7/1
  Hit Crossing8/1 -> Data Type Conversion12/1
  Saturation1/1 -> xForce2/2
  Sum42/1 -> Divide24/2
  Saturation7/1 -> xForce2/1
  Sum9/1 -> Divide9/1
  lambda-s1R/1 -> Divide9/2, Sum9/2
  [LSOLgolgi] -> L SOL golgi delay/1
  Demux8/4 -> [LTAstim]
  L SOL golgi delay/1 -> Sum10/2
  Sum20/1 -> Divide15/2
  [Lhipc] -> Divide15/1
  Sum31/1 -> Divide16/2
  [Rhipc] -> Divide16/1
  [Rnot] -> Data Type Conversion5/1
  Logical Operator/1 -> [Rnot]
  Cast To Double/1 -> Logical Operator4/1
  Logical Operator4/1 -> [Lnot]
  [xRheel] -> noisy8/1(In1)
  [RSOLgolgi] -> R SOL golgi delay/1
  Sum57/1 -> Data Type Conversion2/1
  IsPositive1/1 -> Data Type Conversion3/1
  Sum46/1 -> IsPositive1/1, IsPositive7/1
  IsPositive/1 -> Data Type Conversion8/1
  [Lnot] -> Data Type Conversion10/1
  Gain9/1 -> Sum9/1
  Add8/1 -> Switch2/2, Switch2/1
  L Skin Load Sensor delay6/1 -> Divide7/2, Divide14/1, Add8/2, Compare To Constant4/1
  IsPositive3/1 -> Logical Operator6/1
  IsPositive2/1 -> Logical Operator6/2
  Logical Operator6/1 -> IMsRight/1(right2left)
  IsPositive4/1 -> Logical Operator7/2
  IsPositive5/1 -> Logical Operator7/1
  Logical Operator7/1 -> IMsLeft/4(right2left)
  Switch4/1 -> Hit Crossing7/1
  IsPositive6/1 -> Cast To Double3/1
  IsPositive7/1 -> Cast To Double4/1
  Cast To Double4/1 -> Switch6/1, Switch3/3
  F-S2/1 -> Sum11/2
  F-S6/1 -> Sum40/1
  F-S3/1 -> Sum38/2
  F-S4/1 -> Sum27/1
  noisy6/1(Out1) -> Divide8/1, Divide2/2
  noisy/1(Out1) -> Sum44/2, Sum29/1, Sum46/2, Sum3/2
  Sum21/1 -> Mux1/5, Gain62/1
  Sum16/1 -> Gain4/1, Mux7/1
  Demux8/1 -> [LRFstim]
  Sum15/1 -> Mux8/2, Sum18/2
  motorpoolL4/1 -> Subsystem1/3(In2), Sum37/2
  Subsystem1/1(Out1) -> Sum37/1
  Subsystem1/2(Out2) -> Sum36/2
  motorpoolL3/1 -> Subsystem1/1(In1), Sum36/1
  Demux5/4 -> [RRFstim]
  Sum19/1 -> Mux4/4
  Subsystem4/1(Out1) -> Sum47/1
  motorpoolR3/1 -> Subsystem4/3(In2), Sum47/2
  motorpoolR4/1 -> Subsystem4/1(In1), Sum48/1
  Subsystem4/2(Out2) -> Sum48/2
  Divide24/1 -> Mux6/2
  Gain5/1 -> Sum42/2
  lambda-s1L/1 -> Sum42/1, Divide24/1
  Sum55/1 -> motorpoolR3/2
  AkneeFlexL/1 -> Sum34/2
  Sum34/1 -> motorpoolR4/1
  Sum54/1 -> motorpoolL3/1
  Sum5/1 -> motorpoolL4/2
  AkneeFlexR/1 -> Sum5/2
  Kq1/1 -> Sum30/1
  Sum25/1 -> Sum52/1, Sum53/1
  thetao/1 -> Divide17/2
  [Theta] -> To Workspace7/1, L SOL golgi delay1/1, Mux10/1
  F-S11/1 -> Body Pitch Velocity Sense delay/1
  [dTheta] -> Mux10/2
  Mux10/1 -> Scope/1
  AkneeFlexR1/1 -> Sum5/1
  [Knee_pain] -> knee pain delay/1
  KKneeExt/1 -> noisy4/1(In1)
  AkneeExt/1 -> Sum54/2
  noisy4/1(Out1) -> Sum54/1
  AkneeFlexL1/1 -> Sum34/1
  [KneeR_pain] -> knee pain delay R/1
  KKneeExt1/1 -> noisy11/1(In1)
  AkneeExt1/1 -> Sum55/2
  noisy11/1(Out1) -> Sum55/1
  L Skin Load Sensor delay/1 -> Logical Operator5/2, [Lhipc], Terminator28/1
  Demux11/1 -> Sum53/2
  Sum53/1 -> Kq1/1
  Sum52/1 -> Kq/1
  Demux/1 -> Sum52/2
  [LHipState] -> noisy3/1(In1)
  [RHipState] -> noisy7/1(In1)
  Divide21/1 -> Gain/1
  lambdaxL/1 -> Divide21/1, Sum50/1
  Sum50/1 -> Divide21/2
  lenf_ref/1 -> Sum51/2
  Sum51/1 -> Sum50/2
  Divide9/1 -> Mux14/2
  Divide11/1 -> Mux14/1
  Sum56/1 -> Sum49/2
  lean_ref/1 -> Sum56/2
  L SOL golgi delay1/1 -> Sum51/1, Sum56/1
  Sum49/1 -> Divide11/2
  lambdaxR/1 -> Sum49/1, Divide11/1
  [ux] -> Mux15/3, Mux5/3
  Gain/1 -> Mux6/1
  Data Type Conversion5/1 -> Mux15/7
  Data Type Conversion11/1 -> Mux15/8
  Switch5/1 -> Mux15/5
  Sum13/1 -> motorpoolL6/2
  Data Type Conversion2/1 -> Mux15/6
  Data Type Conversion4/1 -> Mux5/5
  Data Type Conversion7/1 -> Mux5/6
  Data Type Conversion6/1 -> Mux5/7
  Data Type Conversion12/1 -> Mux5/8
  Logical Operator2/1 -> Data Type Conversion4/1
  Hit Crossing/1 -> Logical Operator2/1
  Hit Crossing1/1 -> Logical Operator2/2
  Data Type Conversion3/1 -> Switch3/1, Switch6/3
  Hit Crossing4/1 -> Data Type Conversion6/1
  Data Type Conversion10/1 -> Hit Crossing4/1
  Hit Crossing2/1 -> Sum57/1
  Hit Crossing3/1 -> Sum57/2
  Data Type Conversion13/1 -> Hit Crossing3/1
  [Lhipc] -> Data Type Conversion13/1
  Gain3/1 -> Mux7/5
  Gain4/1 -> Mux7/2
  Sum18/1 -> Mux8/1
  Gain61/1 -> Mux1/1
  Gain62/1 -> Mux1/4
  [balance] -> Mux12/1, Mux11/1, [ConBal]
  Product/1 -> Sum6/1
  KAnkleExt/1 -> Product/1
  Product1/1 -> Sum32/1
  KAnkleFlex1/1 -> Product1/1
  Product2/1 -> Sum13/1
  KAnkleFlex/1 -> Product2/2
  Product3/1 -> Sum35/1
  KAnkleExt1/1 -> Product3/2
  [ConBal] -> Product/2
  [ConBal] -> Product1/2, Product2/1
  [ConBal] -> Product3/1
  knee pain delay/1 -> KKneeExt/1
  knee pain delay R/1 -> KKneeExt1/1
  [us] -> Mux15/2, Mux5/2
  [ub] -> Mux15/1, Mux5/1
  Switch6/1 -> Hit Crossing1/1
  Switch3/1 -> Hit Crossing8/1
  [backgait] -> Divide25/1, Switch8/2, Sum23/1, Sum24/2, Switch4/2, Switch5/2, Mux12/3, Switch7/2, Sum43/1, Switch6/2, Switch3/2, Hit Crossing5/1, Mux11/3
  AHipFlexL1/1 -> IsPositive2/1
  AHipFlexL2/1 -> IsPositive3/1
  Demux23/5 -> motorpoolL5/2
  Sum24/1 -> Hit Crossing2/1
  Data Type Conversion8/1 -> Switch4/1, Switch5/3
  Cast To Double3/1 -> Switch5/1, Switch4/3
  thetabo/1 -> Divide25/2
  Divide17/1 -> Sum25/1
  Divide25/1 -> Sum25/2
  Sum43/1 -> Subsystem2/2(m), Subsystem1/2(m), Subsystem3/2(m)
  Sum23/1 -> Subsystem6/2(m), Subsystem4/2(m), Subsystem5/2(m)
  Switch7/1 -> Sum46/1
  Switch8/1 -> Sum44/1
  Data Type Conversion9/1 -> Mux5/4
  Logical Operator5/1 -> Data Type Conversion9/1
  Hit Crossing5/1 -> Logical Operator5/1
  Mux12/1 -> IMsRight/2(drivers)
  [gait] -> Sum43/2, Hit Crossing/1, Mux11/2, Divide17/1, Sum23/2, Mux12/2, Sum24/1
  IMsLeft/1(beta) -> Demux23/1
  Demux23/1 -> motorpoolL1/2
  Demux23/2 -> motorpoolL2/1
  Demux23/3 -> motorpoolL3/2
  Demux23/4 -> motorpoolL4/1
  Demux23/6 -> motorpoolL6/1
  IMsRight/1(beta) -> Demux6/1
  AHipFlexL3/1 -> IsPositive5/1
  AHipFlexL4/1 -> IsPositive4/1
  Demux6/1 -> motorpoolR1/1
  Demux6/3 -> motorpoolR3/1
  Demux6/5 -> motorpoolR5/1
  Demux6/2 -> motorpoolR2/2
  Demux6/4 -> motorpoolR4/2
  Demux6/6 -> motorpoolR6/2
  Demux3/1 -> Terminator1/1
  Demux3/2 -> Terminator2/1
